simulink model "OBC"  (R2023a)
settings: Solver=VariableStepAuto  StartTime=0.0  StopTime=10.0  RelTol=1e-3
settings Model: DataDictionary=SatelliteTelescope.sldd  Creator=Ren4  LastModifiedBy=Ren4

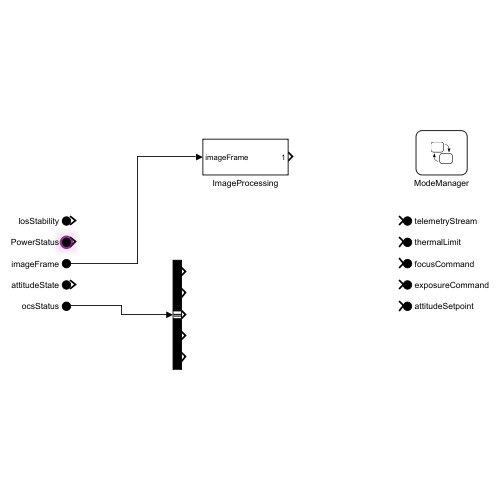
[thumbnail: Simulink's stored preview of the top-level diagram]
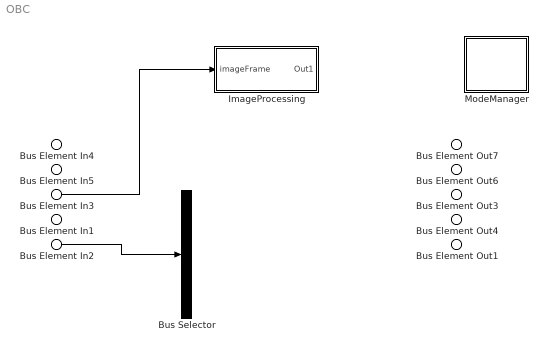
== system OBC ==
  Bus Element In4 : Inport  PortName=losStability
  Bus Element In5 : Inport  Port=2  PortName=PowerStatus
  Bus Element In3 : Inport  Port=3  PortName=imageFrame
  Bus Element In1 : Inport  Port=4  PortName=attitudeState
  Bus Element In2 : Inport  Port=5  PortName=ocsStatus
  Bus Selector : BusSelector  OutputSignals=wheelHealth,gyroHealth,starTrackerHealth,faultCode,mode
  ImageProcessing : Subsystem
  ModeManager : Stateflow chart  TreatAsAtomicUnit=on
  Bus Element Out7 : Outport  PortName=telemetryStream
  Bus Element Out6 : Outport  Port=2  PortName=thermalLimit
  Bus Element Out3 : Outport  Port=3  PortName=focusCommand
  Bus Element Out4 : Outport  Port=4  PortName=exposureCommand
  Bus Element Out1 : Outport  Port=5  PortName=attitudeSetpoint
  wires:
  Bus Element In3/1 -> ImageProcessing/1(imageFrame)
  Bus Element In2/1 -> Bus Selector/1

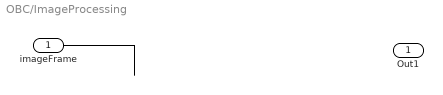
== system OBC/ImageProcessing ==
  imageFrame : Inport
  Out1 : Outport
  wires:
  imageFrame/1 -> ?

== stateflow chart OBC/ModeManager ==
  state Image
  state Transmit
  state Diagnostic
  state StandBy
  (default) -> Image
